simulink model "DSimulator_abbIRB4HP_JPIDAda"  (R2023b)
settings: Solver=ode1  StartTime=0.0  StopTime=75  FixedStep=0.001  RelTol=1e-3  EnableMultiTasking=on
values from neighbouring files (symbols this model uses):
  g = 9.81    [run_abb_irb120_JPIDAda.m]
undefined symbols (not defined in the file or in its folder): Dinamic_abbIRB4HP, plotRobotJAda, Qpr_abbIRB4, Sq_abbIRB4, tauAdaptivePIDR, thetaHatDot_abbIRB4, trajGen_abbIRB4, Yr_abbIRB4
CloseFcn:
  | EraseHandles
Description:
  | This model simualtes the robot ABB IRB-120 (4DOF) with a P(I)D-like controller with robot regressor.
settings Model: Creator=E. Dean  LastModifiedBy=ellio
settings SolverCC: ConcurrentTasks=on  AlgebraicLoopSolver=TrustRegion
settings DataIOCC: LimitDataPoints=on  SaveFormat=Array  SignalLoggingSaveFormat=ModelDataLogs  ReturnWorkspaceOutputs=off
settings OptimizationCC: ExpressionDepthLimit=2147483647  LifeSpan=inf
settings DebuggingCC: UnderspecifiedInitializationDetection=Classic  MergeDetectMultiDrivingBlocksExec=none  SolverPrmCheckMsg=warning  FcnCallInpInsideContextMsg=warning  UnconnectedInputMsg=warning  UnconnectedOutputMsg=warning  UnconnectedLineMsg=warning  StateNameClashWarn=warning  SFUnexpectedBacktrackingDiag=warning  SFNoUnconditionalDefaultTransitionDiag=warning  SFExecutionAtInitializationDiag=none  ArithmeticOperatorsInVariantConditions=warning
settings HardwareCC: ProdBitPerPointer=32  ProdBitPerSizeT=32  ProdBitPerPtrDiffT=32  ProdLargestAtomicFloat=None  ProdIntDivRoundTo=Undefined  ProdEndianess=Unspecified  ProdWordSize=32  ProdHWDeviceType=32-bit Generic
settings ModelReferenceCC: EnableRefExpFcnMdlSchedulingChecks=on  PropagateSignalLabelsOutOfModel=off
settings SFSimCC: SimUseLocalCustomCode=off  CustomCodeUndefinedFunction=UseInterfaceOnly
settings RTWCC: RTWUseLocalCustomCode=off  DLArmComputeVersion=19.05
settings CodeAppCC: StateflowObjectComments=on
settings GRTTargetCC: TargetLangStandard=C89/C90 (ANSI)  CombineOutputUpdateFcns=off  GRTInterface=on
settings ConfigComp: CovMetricSettings=dw  CovSaveCumulativeToWorkspaceVar=on  CovSaveSingleToWorkspaceVar=on

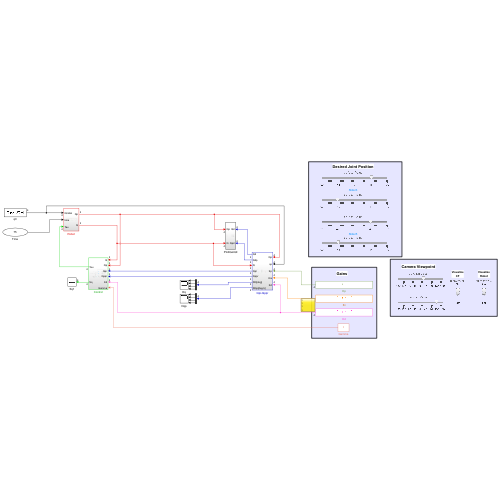
[thumbnail: Simulink's stored preview of the top-level diagram]
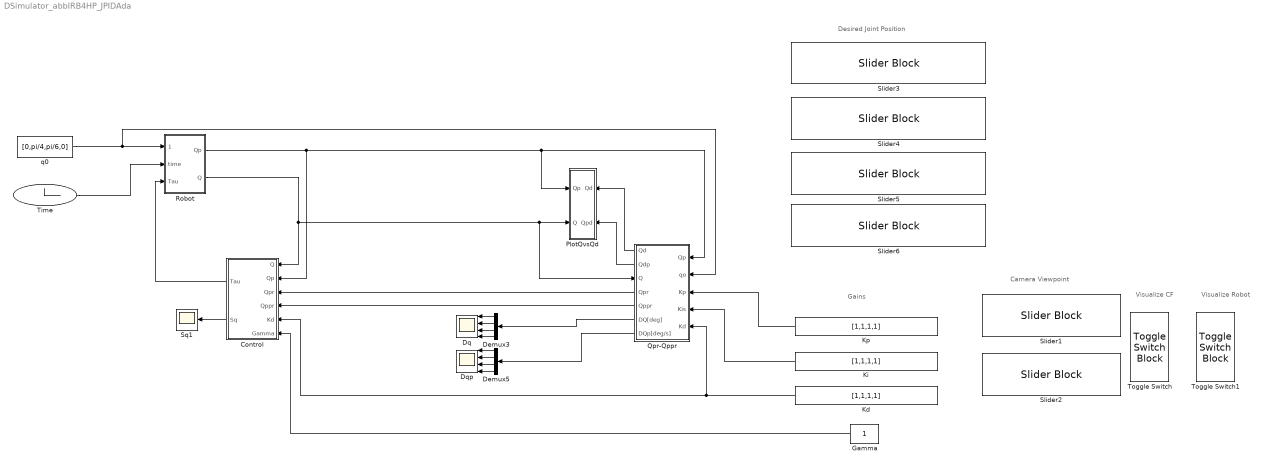
== system DSimulator_abbIRB4HP_JPIDAda ==
  note: Gains
  note: Visualize
      | CF
  note: Desired Joint Position
  note: Camera Viewpoint
  note: Visualize
      | Robot
  Control : Subsystem
  Demux3 : Demux
  Demux5 : Demux
  Dq : Scope  NumInputPorts=4
  Dqp : Scope  NumInputPorts=4
  Gamma : Constant
  Kd : Constant  Value=[1,1,1,1]
  Ki : Constant  Value=[1,1,1,1]
  Kp : Constant  Value=[1,1,1,1]
  PlotQvsQd : Subsystem
      settings: PortSchema="{\"entries\":[{\"content\":{\"sides\":[{\"content\":{\"connectorIds\":[\"In1\",\"In2\"]},\"type\":\"ConnectorPlacement.EquallySpacedRectSide\",\"uuid\":\"0ee6224f-6764-463a-9bad-8b013ba062e4\"},{\"content\":{\"connectorIds\":[\"In3\",\"In4\"],\"side\":\"RIGHT\"},\"type\":\"ConnectorPlacement.EquallySpacedRectSide\",\"uuid\":\"0aa5cc1a-1f9a-4b91-a80f-0f5a47f21dc5\"},{\"content\":{\"connectorIds\":[],\"side\":\"TOP\"},\"type\":\"ConnectorPlacement.EquallySpacedRectSide\",\"uuid\":\"0621933a-b21a-4d17-bd2c-a4a6b51319e2\"}]},\"type\":\"ConnectorPlacement.EquallySpacedConnector\",\"uuid\":\"178ee6f9-8179-4351-91f8-4db33d3c7c28\"}],\"packageUris\":[\"http://schema.mathworks.com/mf0/Connector/R2020b\"],\"version\":\"1.0\"}"
  Qpr-Qppr : Subsystem
      settings: PortSchema="{\"entries\":[{\"content\":{\"sides\":[{\"content\":{\"connectorIds\":[\"In1\",\"In2\",\"In3\",\"In4\",\"In5\"]},\"type\":\"ConnectorPlacement.EquallySpacedRectSide\",\"uuid\":\"7dbdf085-398c-44a0-9fac-a1aff608b1f8\"},{\"content\":{\"connectorIds\":[\"Out1\",\"Out2\",\"In6\",\"Out3\",\"Out4\",\"Out5\",\"Out6\"],\"side\":\"RIGHT\"},\"type\":\"ConnectorPlacement.EquallySpacedRectSide\",\"uuid\":\"148c2c27-15e0-4cef-94d9-b1afb135f7fd\"},{\"content\":{\"connectorIds\":[],\"side\":\"TOP\"},\"type\":\"ConnectorPlacement.EquallySpacedRectSide\",\"uuid\":\"5241d212-3439-41c2-ba91-8c6bc4af1e12\"}]},\"type\":\"ConnectorPlacement.EquallySpacedConnector\",\"uuid\":\"9b119900-6e6c-418f-b24a-88dd51a30d73\"}],\"packageUris\":[\"http://schema.mathworks.com/mf0/Connector/R2020b\"],\"version\":\"1.0\"}"
  Robot : Subsystem
  Slider1 : SliderBlock  ScaleMin=-180  ScaleMax=180  TickInterval=45
  Slider2 : SliderBlock  ScaleMin=-180  ScaleMax=180  TickInterval=45
  Slider{3..6} (4 alike) : SliderBlock  ScaleMin=-90  ScaleMax=90  TickInterval=45
  Sq1 : Scope
  Time : Clock
  Toggle Switch : ToggleSwitchBlock
      settings: Values={{'Off', 'On'}, [0 1]}
  Toggle Switch1 : ToggleSwitchBlock
      settings: Values={{'Off', 'On'}, [0 1]}
  q0 : Constant  Value=[0,pi/4,pi/6,0]
  wires:
  Demux3/2 -> Dq/2
  Demux3/1 -> Dq/1
  Demux3/3 -> Dq/3
  Demux3/4 -> Dq/4
  Kd/1 -> Control/5(Kd), Qpr-Qppr/5(Kd)
  Demux5/1 -> Dqp/1
  Demux5/4 -> Dqp/4
  Demux5/3 -> Dqp/3
  Demux5/2 -> Dqp/2
  Kp/1 -> Qpr-Qppr/3(Kp)
  Ki/1 -> Qpr-Qppr/4(Kis)
  Qpr-Qppr/5(DQ[deg]) -> Demux3/1
  Qpr-Qppr/6(DQp[deg/s]) -> Demux5/1
  Qpr-Qppr/1(Qd) -> PlotQvsQd/3(Qd)
  Qpr-Qppr/2(Qdp) -> PlotQvsQd/4(Qpd)
  Qpr-Qppr/3(Qpr) -> Control/3(Qpr)
  Qpr-Qppr/4(Qppr) -> Control/4(Qppr)
  Control/2(Sq) -> Sq1/1
  Robot/2(Q) -> Qpr-Qppr/6(Q), PlotQvsQd/2(Q), Control/1(Q)
  Robot/1(Qp) -> Qpr-Qppr/1(Qp), PlotQvsQd/1(Qp), Control/2(Qp)
  q0/1 -> Qpr-Qppr/2(qo), Robot/1(Qinitial)
  Time/1 -> Robot/2(time)
  Control/1(Tau) -> Robot/3(Tau)
  Gamma/1 -> Control/6(Gamma)

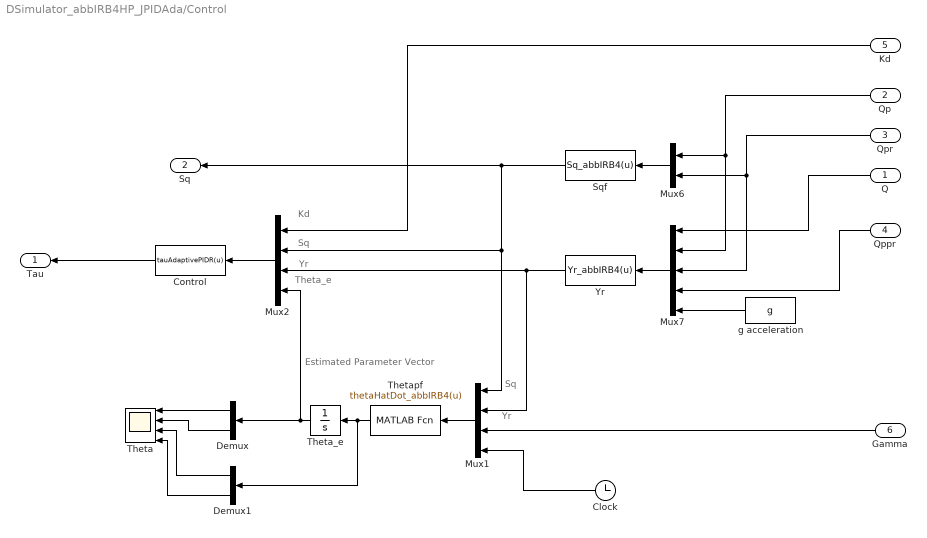
== system DSimulator_abbIRB4HP_JPIDAda/Control ==
  note: Theta_e
  note: Yr
  note: Sq
  note: Kd
  note: Estimated
      | Parameter
      | Vector
  note: Yr
  note: Sq
  Q : Inport
  Qp : Inport  Port=2
  Qpr : Inport  Port=3
  Qppr : Inport  Port=4
  Kd : Inport  Port=5
  Gamma : Inport  Port=6
  Clock : Clock
  Control : MATLABFcn  MATLABFcn=tauAdaptivePIDR(u)  OutputDimensions=4
  Demux : Demux  Outputs=2
  Demux1 : Demux  Outputs=2
  Mux1 : Mux
  Mux2 : Mux
  Mux6 : Mux  Inputs=2
  Mux7 : Mux  Inputs=5
  Sqf : MATLABFcn  MATLABFcn=Sq_abbIRB4(u)  OutputDimensions=4
  Theta : Scope  NumInputPorts=4
  Theta_e : Integrator
  Thetapf : MATLABFcn  MATLABFcn=thetaHatDot_abbIRB4(u)  OutputDimensions=39
  Yr : MATLABFcn  MATLABFcn=Yr_abbIRB4(u)  OutputDimensions=4*39
  g acceleration : Constant  Value=g
  Tau : Outport
  Sq : Outport  Port=2
  wires:
  Yr/1 -> Mux1/2, Mux2/3
  g acceleration/1 -> Mux7/5
  Qpr/1 -> Mux7/3, Mux6/2
  Qppr/1 -> Mux7/4
  Mux7/1 -> Yr/1
  Mux6/1 -> Sqf/1
  Mux2/1 -> Control/1
  Qp/1 -> Mux7/2, Mux6/1
  Kd/1 -> Mux2/1
  Control/1 -> Tau/1
  Q/1 -> Mux7/1
  Sqf/1 -> Sq/1, Mux2/2, Mux1/1
  Mux1/1 -> Thetapf/1
  Gamma/1 -> Mux1/3
  Clock/1 -> Mux1/4
  Thetapf/1 -> Demux1/1, Theta_e/1
  Theta_e/1 -> Demux/1, Mux2/4
  Demux/1 -> Theta/1
  Demux/2 -> Theta/2
  Demux1/1 -> Theta/3
  Demux1/2 -> Theta/4

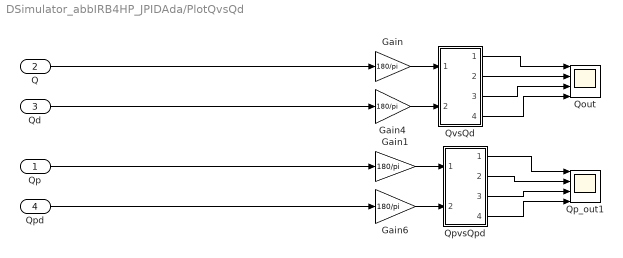
== system DSimulator_abbIRB4HP_JPIDAda/PlotQvsQd ==
  Qp : Inport
  Q : Inport  Port=2
  Qd : Inport  Port=3
  Qpd : Inport  Port=4
  Gain{,1,4,6} (4 alike) : Gain  Gain=180/pi
  Qout : Scope  NumInputPorts=4
  Qp_out1 : Scope  NumInputPorts=4
  QpvsQpd : Subsystem
  QvsQd : Subsystem
  wires:
  QvsQd/2(q2o) -> Qout/2
  Qd/1 -> Gain4/1
  QvsQd/3(q3o) -> Qout/3
  QpvsQpd/2(qp2o) -> Qp_out1/2
  Qp/1 -> Gain1/1
  Gain/1 -> QvsQd/1(In1)
  Gain1/1 -> QpvsQpd/1(In1)
  QpvsQpd/3(qp3o) -> Qp_out1/3
  Qpd/1 -> Gain6/1
  Q/1 -> Gain/1
  Gain4/1 -> QvsQd/2(In2)
  QpvsQpd/4(qp4o) -> Qp_out1/4
  QpvsQpd/1(qp1o) -> Qp_out1/1
  QvsQd/1(q1o) -> Qout/1
  QvsQd/4(q4o) -> Qout/4
  Gain6/1 -> QpvsQpd/2(In2)

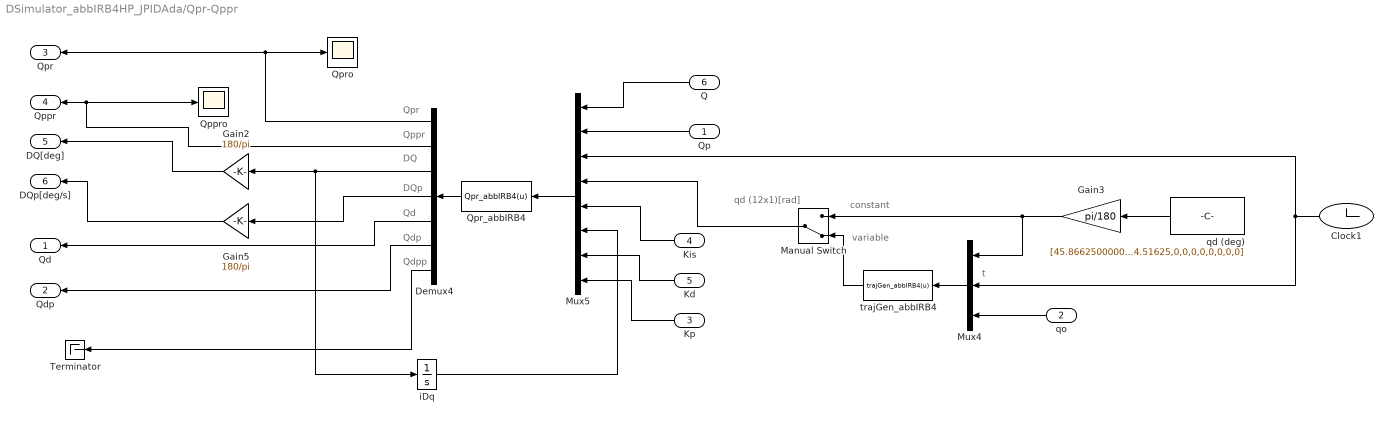
== system DSimulator_abbIRB4HP_JPIDAda/Qpr-Qppr ==
  note: Qdpp
  note: Qpr
  note: variable
  note: constant
  note: t
  note: qd (12x1)[rad]
  note: DQ
  note: DQp
  note: Qd
  note: Qdp
  note: Qppr
  Qp : Inport
  qo : Inport  Port=2
  Kp : Inport  Port=3
  Kis : Inport  Port=4
  Kd : Inport  Port=5
  Q : Inport  Port=6
  Clock1 : Clock
  Demux4 : Demux  Outputs=7
  Gain2 : Gain  Gain=180/pi
  Gain3 : Gain  Gain=pi/180
  Gain5 : Gain  Gain=180/pi
  Manual Switch : ManualSwitch  CurrentSetting=0
  Mux4 : Mux  Inputs=3
  Mux5 : Mux  Inputs=8
  Qppro : Scope
  Qpr_abbIRB4 : MATLABFcn  MATLABFcn=Qpr_abbIRB4(u)  OutputDimensions=28
  Qpro : Scope
  Terminator : Terminator
  iDq : Integrator
  qd (deg) : Constant  Value=[45.86625000000001,-46.67625,44.04374999999999,-44.51625,0,0,0,0,0,0,0,0]
  trajGen_abbIRB4 : MATLABFcn  MATLABFcn=trajGen_abbIRB4(u)  OutputDimensions=12
  Qd : Outport
  Qdp : Outport  Port=2
  Qpr : Outport  Port=3
  Qppr : Outport  Port=4
  DQ[deg] : Outport  Port=5
  DQp[deg/s] : Outport  Port=6
  wires:
  Mux4/1 -> trajGen_abbIRB4/1
  Mux5/1 -> Qpr_abbIRB4/1
  Demux4/7 -> Terminator/1
  iDq/1 -> Mux5/6
  qd (deg)/1 -> Gain3/1
  Gain5/1 -> DQp[deg/s]/1
  Kis/1 -> Mux5/5
  Gain2/1 -> DQ[deg]/1
  Demux4/4 -> Gain5/1
  Demux4/1 -> Qpro/1, Qpr/1
  Kp/1 -> Mux5/8
  Qp/1 -> Mux5/2
  trajGen_abbIRB4/1 -> Manual Switch/2
  Q/1 -> Mux5/1
  Demux4/2 -> Qppro/1, Qppr/1
  Kd/1 -> Mux5/7
  Demux4/3 -> Gain2/1, iDq/1
  Qpr_abbIRB4/1 -> Demux4/1
  Clock1/1 -> Mux5/3, Mux4/2
  Manual Switch/1 -> Mux5/4
  Demux4/5 -> Qd/1
  Demux4/6 -> Qdp/1
  Gain3/1 -> Mux4/1, Manual Switch/1
  qo/1 -> Mux4/3

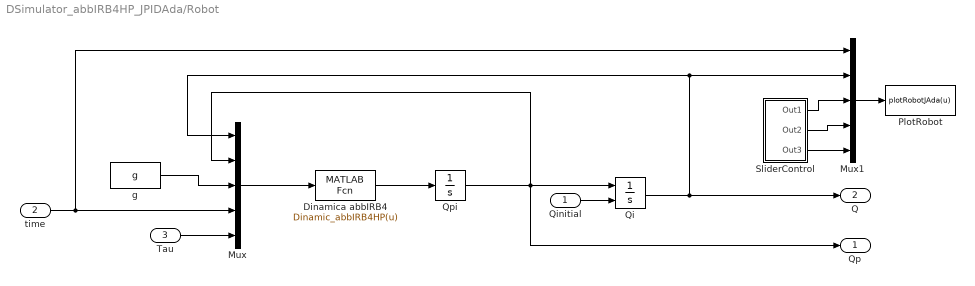
== system DSimulator_abbIRB4HP_JPIDAda/Robot ==
  Qinitial : Inport
  time : Inport  Port=2
  Tau : Inport  Port=3
  Dinamica abbIRB4 : MATLABFcn  MATLABFcn=Dinamic_abbIRB4HP(u)  OutputDimensions=4
  Mux : Mux  Inputs=5
  Mux1 : Mux  Inputs=5
  PlotRobot : MATLABFcn  MATLABFcn=plotRobotJAda(u)  OutputDimensions=0
  Qi : Integrator  InitialConditionSource=external  InitialCondition=[0;0;0;0]
  Qpi : Integrator  InitialCondition=[0;0;0;0]
  SliderControl : Subsystem
  g : Constant  Value=g
  Qp : Outport
  Q : Outport  Port=2
  wires:
  SliderControl/2(Out2) -> Mux1/4
  g/1 -> Mux/3
  Qpi/1 -> Qp/1, Qi/1, Mux/2
  Dinamica abbIRB4/1 -> Qpi/1
  Mux1/1 -> PlotRobot/1
  Mux/1 -> Dinamica abbIRB4/1
  time/1 -> Mux1/1, Mux/4
  Tau/1 -> Mux/5
  Qi/1 -> Q/1, Mux1/2, Mux/1
  Qinitial/1 -> Qi/2
  SliderControl/1(Out1) -> Mux1/3
  SliderControl/3(Out3) -> Mux1/5

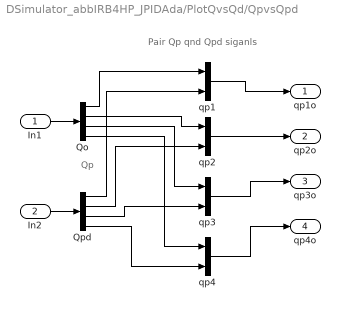
== system DSimulator_abbIRB4HP_JPIDAda/PlotQvsQd/QpvsQpd ==
  note: Qp
  note: Pair Qp qnd Qpd siganls
  In1 : Inport
  In2 : Inport  Port=2
  Qo : Demux
  Qpd : Demux
  qp{1..4} (4 alike) : Mux  Inputs=2
  qp1o : Outport
  qp2o : Outport  Port=2
  qp3o : Outport  Port=3
  qp4o : Outport  Port=4
  wires:
  Qpd/1 -> qp1/2
  Qpd/2 -> qp2/2
  Qpd/4 -> qp4/2
  Qo/4 -> qp4/1
  Qo/3 -> qp3/1
  Qo/1 -> qp1/1
  In1/1 -> Qo/1
  qp2/1 -> qp2o/1
  In2/1 -> Qpd/1
  qp4/1 -> qp4o/1
  qp1/1 -> qp1o/1
  Qo/2 -> qp2/1
  qp3/1 -> qp3o/1
  Qpd/3 -> qp3/2

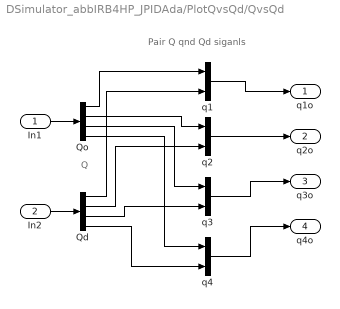
== system DSimulator_abbIRB4HP_JPIDAda/PlotQvsQd/QvsQd ==
  note: Q
  note: Pair Q qnd Qd siganls
  In1 : Inport
  In2 : Inport  Port=2
  Qd : Demux
  Qo : Demux
  q{1..4} (4 alike) : Mux  Inputs=2
  q1o : Outport
  q2o : Outport  Port=2
  q3o : Outport  Port=3
  q4o : Outport  Port=4
  wires:
  Qd/1 -> q1/2
  Qd/2 -> q2/2
  Qd/4 -> q4/2
  Qo/4 -> q4/1
  Qo/3 -> q3/1
  Qo/1 -> q1/1
  In1/1 -> Qo/1
  q2/1 -> q2o/1
  In2/1 -> Qd/1
  q4/1 -> q4o/1
  q1/1 -> q1o/1
  Qo/2 -> q2/1
  q3/1 -> q3o/1
  Qd/3 -> q3/2

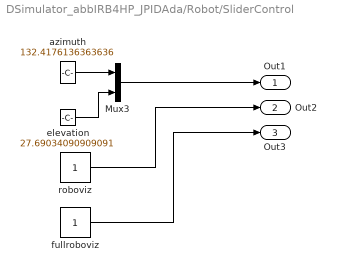
== system DSimulator_abbIRB4HP_JPIDAda/Robot/SliderControl ==
  Mux3 : Mux  Inputs=2
  azimuth : Constant  Value=132.4176136363636
  elevation : Constant  Value=27.69034090909091
  fullroboviz : Constant
  roboviz : Constant
  Out1 : Outport
  Out2 : Outport  Port=2
  Out3 : Outport  Port=3
  wires:
  azimuth/1 -> Mux3/1
  roboviz/1 -> Out2/1
  elevation/1 -> Mux3/2
  Mux3/1 -> Out1/1
  fullroboviz/1 -> Out3/1
